simulink model "probeModel"  (R2015b)
settings: Solver=VariableStepAuto  SolverMode=SingleTasking  StartTime=0.0  StopTime=10.0  RelTol=1e-3
libraries: simulink x1, probeLib x1
Description:
  | Model description line 1
  | line 2
settings Model: ModifiedByFormat=matlabdomain  Creator=matlabdomain  LastModifiedBy=matlabdomain
settings DataIOCC: LimitDataPoints=off  ReturnWorkspaceOutputs=on
settings DebuggingCC: UnconnectedInputMsg=none  UnconnectedOutputMsg=none  UnconnectedLineMsg=none  AllowSymbolicDim=on  SFUnexpectedBacktrackingDiag=error  SFNoUnconditionalDefaultTransitionDiag=error
settings ModelReferenceCC: UpdateModelReferenceTargets=IfOutOfDate  EnableRefExpFcnMdlSchedulingChecks=off  PropagateSignalLabelsOutOfModel=on
settings SFSimCC: SimUseLocalCustomCode=on
settings RTWCC: RTWUseLocalCustomCode=on
settings GRTTargetCC: TargetLangStandard=C99 (ISO)
settings ConfigComp: CovMetricSettings=de  CovSaveCumulativeToWorkspaceVar=off  CovSaveSingleToWorkspaceVar=off  CovModelRefEnable=Off  CovExternalEMLEnable=on  CovBoundaryAbsTol=1.0e-5

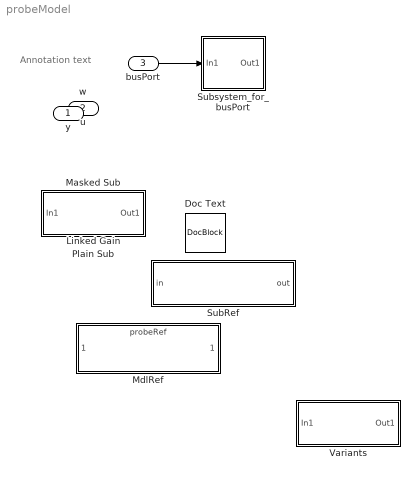
== system probeModel ==
  note: Annotation text
  u : Inport  Description=input u doc  OutDataTypeStr=double  PortDimensions=3
  w : Inport  Description=second input  Port=2
  busPort : Inport  Port=3
  Doc Text : simulink/Model-Wide Utilities/DocBlock  DocumentType=Text
      content=|
      | DocBlock text content.
  Linked Gain : probeLib/Gain Block  gain=2  mode=fast  flag=on
  Masked Sub : Subsystem  mask(ModelMaskType){gain=2, mode=fast, flag=on}
      mask prompts: gain "Gain value"; flag "Enable"
      mask help: Masked subsystem in model.
      mask Help: Masked help in model.
      mask TypeOptions mode: fast | slow
  MdlRef : ModelReference  ModelNameDialog=probeRef  SimulationMode=Normal  ModelReferenceVersion=1.1
  Plain Sub : Subsystem  Description=Plain subsystem description
  SubRef : Subsystem  mask(SubFileMaskType){k=1}
      mask prompts: k "Factor k"
      mask help: Subsystem file mask description
      mask Help: Subsystem file mask help
  Subsystem_for_busPort : Subsystem
  Variants : Subsystem  Variant=on
  y : Outport  Description=output y doc
  wires:
  busPort/1 -> Subsystem_for_busPort/1(In1)

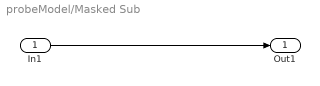
== system probeModel/Masked Sub ==
  In1 : Inport
  Out1 : Outport
  wires:
  In1/1 -> Out1/1

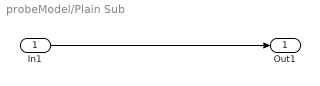
== system probeModel/Plain Sub ==
  In1 : Inport
  Out1 : Outport
  wires:
  In1/1 -> Out1/1

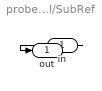
== system probeModel/SubRef ==
  in : Inport  Description=sub input doc  OutDataTypeStr=single
  out : Outport
  wires:
  in/1 -> out/1

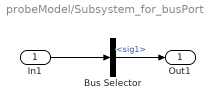
== system probeModel/Subsystem_for_busPort ==
  In1 : Inport
  Bus Selector : BusSelector  OutputSignals=sig1
  Out1 : Outport
  wires:
  In1/1 -> Bus Selector/1
  Bus Selector/1 -> Out1/1  "<sig1>"

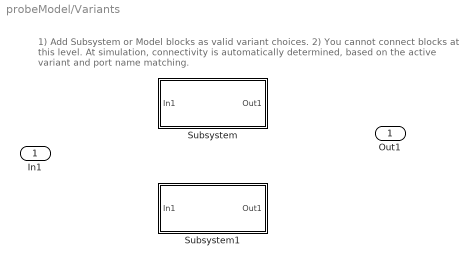
== system probeModel/Variants ==
  note: 1) Add Subsystem or Model blocks as valid variant choices.
      | 2) You cannot connect blocks at this level. At simulation, connectivity is automatically
      | determined, based on the active variant and port name matching.
  In1 : Inport
  Subsystem : Subsystem  VariantControl=true
  Subsystem1 : Subsystem  VariantControl=false
  Out1 : Outport

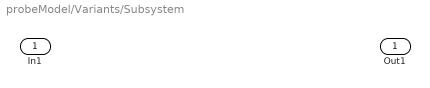
== system probeModel/Variants/Subsystem ==
  In1 : Inport
  Out1 : Outport

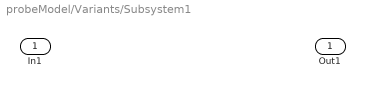
== system probeModel/Variants/Subsystem1 ==
  In1 : Inport
  Out1 : Outport
